simulink model "poly_Traj_lab"  (R2023b)
settings: Solver=VariableStepAuto  StartTime=0.0  StopTime=10.0  RelTol=1e-3
undefined symbols (not defined in the file or in its folder): X, Y, Z
libraries: sm_lib x16, nesl_utility x5, robotcorelib x2, robotmaniplib x1
settings Model: Creator=root  LastModifiedBy=root

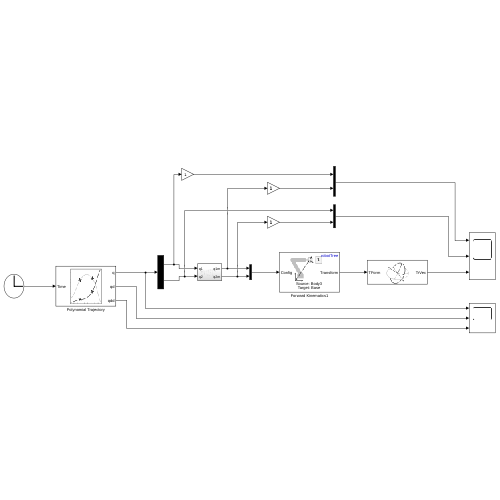
[thumbnail: Simulink's stored preview of the top-level diagram]
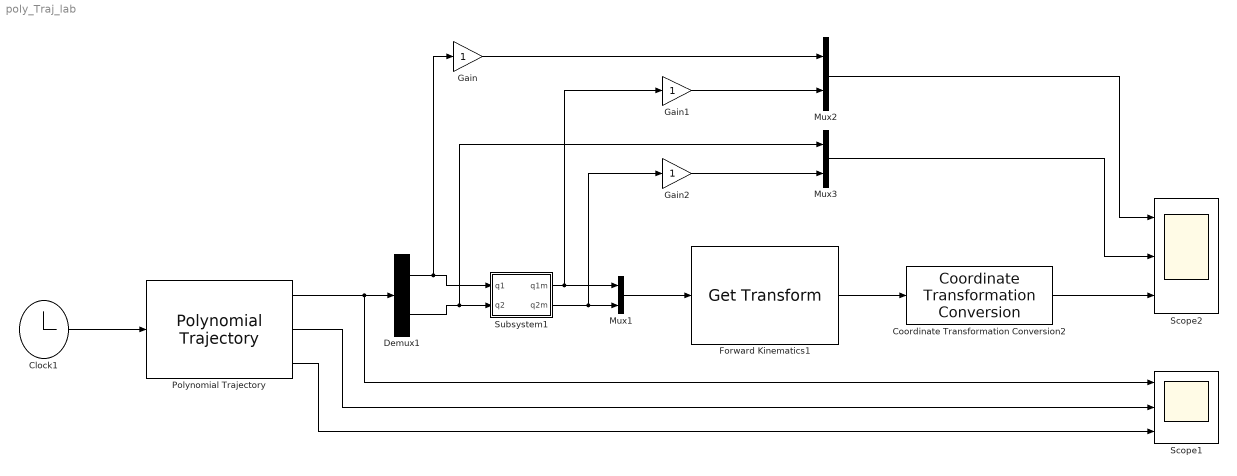
== system poly_Traj_lab ==
  Clock1 : Clock
  Coordinate Transformation Conversion2 : robotcorelib/Coordinate Transformation Conversion  InputRepresentation=Homogeneous Transformation  InputEulerSequence=ZYX  ShowTrVecInputPort=on  OutputRepresentation=Translation Vector  OutputEulerSequence=ZYX  ShowTrVecOutputPort=on  SimulateUsing=Interpreted execution
      settings: LibrarySourceBlock=navlib/Utilities/Coordinate Transformation Conversion
  Demux1 : Demux  Outputs=2
  Forward Kinematics1 : robotmaniplib/Get Transform  RigidBodyTree=robotTree  SourceBody=Body3  TargetBody=Base  SimulateUsing=Interpreted execution
  Gain : Gain
  Gain1 : Gain
  Gain2 : Gain
  Mux1 : Mux  Inputs=2
  Mux2 : Mux  Inputs=2
  Mux3 : Mux  Inputs=2
  Polynomial Trajectory : robotcorelib/Polynomial Trajectory  WaypointSource=Internal  Waypoints=[0 0 pi/2 pi/2; 0 0 -2*pi -2*pi]  TimePoints=[0 2 8 10]  TimeInterval=[ 1, 4 ]  Method=Cubic Polynomial  ParameterSource=Internal  VelocityBoundaryCondition=[0 0 0 0; 0 0 0 0]  AccelerationBoundaryCondition=zeros( 2, 5 )  SimulateUsing=Interpreted execution
  Scope1 : Scope  NumInputPorts=3
  Scope2 : Scope  NumInputPorts=3
  Subsystem1 : Subsystem
  wires:
  Polynomial Trajectory/2 -> Scope1/2
  Demux1/1 -> Gain/1, Subsystem1/1(q1)
  Forward Kinematics1/1 -> Coordinate Transformation Conversion2/1
  Demux1/2 -> Mux3/1, Subsystem1/2(q2)
  Clock1/1 -> Polynomial Trajectory/1
  Mux1/1 -> Forward Kinematics1/1
  Mux2/1 -> Scope2/1
  Coordinate Transformation Conversion2/1 -> Scope2/3
  Mux3/1 -> Scope2/2
  Gain2/1 -> Mux3/2
  Polynomial Trajectory/3 -> Scope1/3
  Subsystem1/2(q2m) -> Gain2/1, Mux1/2
  Gain/1 -> Mux2/1
  Gain1/1 -> Mux2/2
  Polynomial Trajectory/1 -> Scope1/1, Demux1/1
  Subsystem1/1(q1m) -> Gain1/1, Mux1/1

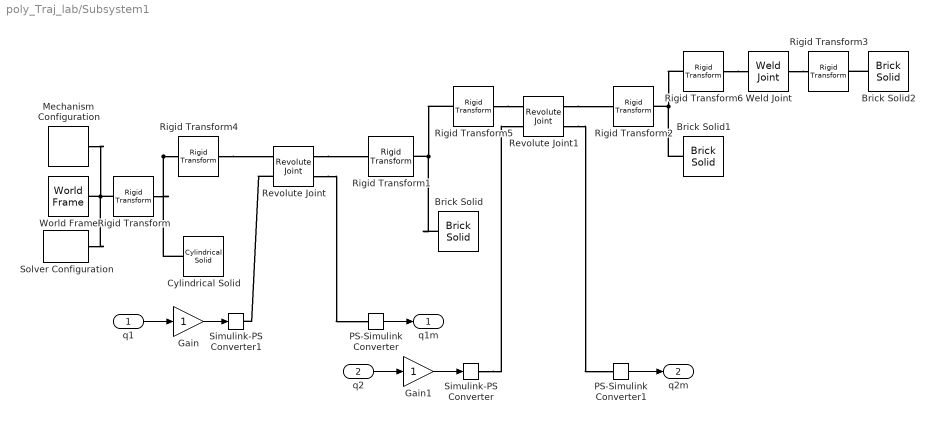
== system poly_Traj_lab/Subsystem1 ==
  q1 : Inport
  q2 : Inport  Port=2
  Brick Solid : sm_lib/Body Elements/Brick Solid  GraphicAmbientColor=[0.15 0.15 0.15 1.0]  BasedOnType=Density  BrickDimensions=[0.6 0.1 0.05]  BrickDimensionsUnits=m  CenterOfMass=[0 0 0]  CenterOfMassUnits=m  GraphicDiffuseColor=[1 0 0]  Density=1000  DensityUnits=kg/m^3  DoExposeReferenceFrame=on  GraphicEmissiveColor=[0.0 0.0 0.0 1.0]  ExportEntireGeometry=off  SerializedFrames=<Frames><Frame><Id>Frame1</Id><Value><Name>F1</Name><Origin><Source>GeometricFeature</Source><FeatureName>+x surface</FeatureName></Origin><PrimaryAxis><DefinedDirection>+Z</DefinedDirection><Source>ReferenceFrame</Source><SourceDirection>+Z</SourceDirection><FeatureName></FeatureName></PrimaryAxis><SecondaryAxis><DefinedDirection>+X</DefinedDirection><Source>ReferenceFrame</Source><SourceDirection>+X</SourceDirection><FeatureName></FeatureName></SecondaryAxis></Value></Frame></Frames>  MarkerShape=Sphere  MarkerSize=10  GraphicType=FromGeometry  InertiaType=CalculateFromGeometry  Mass=1  MassUnits=kg  MomentsOfInertia=[1 1 1]  MomentsOfInertiaUnits=kg*m^2  GraphicOpacity=1.0  ProductsOfInertia=[0 0 0]  ProductsOfInertiaUnits=kg*m^2  GraphicShininess=75  GraphicSpecularColor=[0.5 0.5 0.5 1.0]  GraphicVisPropType=SimpleVisualProperties
  Brick Solid1 : sm_lib/Body Elements/Brick Solid  GraphicAmbientColor=[0.15 0.15 0.15 1.0]  BasedOnType=Density  BrickDimensions=[0.4 0.1 0.05]  BrickDimensionsUnits=m  CenterOfMass=[0 0 0]  CenterOfMassUnits=m  GraphicDiffuseColor=[0 1 0]  Density=1000  DensityUnits=kg/m^3  DoExposeReferenceFrame=on  GraphicEmissiveColor=[0.0 0.0 0.0 1.0]  ExportEntireGeometry=off  SerializedFrames=<Frames><Frame><Id>Frame1</Id><Value><Name>F1</Name><Origin><Source>GeometricFeature</Source><FeatureName>+x surface</FeatureName></Origin><PrimaryAxis><DefinedDirection>+Z</DefinedDirection><Source>ReferenceFrame</Source><SourceDirection>+Z</SourceDirection><FeatureName></FeatureName></PrimaryAxis><SecondaryAxis><DefinedDirection>+X</DefinedDirection><Source>ReferenceFrame</Source><SourceDirection>+X</SourceDirection><FeatureName></FeatureName></SecondaryAxis></Value></Frame></Frames>  MarkerShape=Sphere  MarkerSize=10  GraphicType=FromGeometry  InertiaType=CalculateFromGeometry  Mass=1  MassUnits=kg  MomentsOfInertia=[1 1 1]  MomentsOfInertiaUnits=kg*m^2  GraphicOpacity=1.0  ProductsOfInertia=[0 0 0]  ProductsOfInertiaUnits=kg*m^2  GraphicShininess=75  GraphicSpecularColor=[0.5 0.5 0.5 1.0]  GraphicVisPropType=SimpleVisualProperties
  Brick Solid2 : sm_lib/Body Elements/Brick Solid  GraphicAmbientColor=[0.15 0.15 0.15 1.0]  BasedOnType=Density  BrickDimensions=[0.02 0.02 0.02]  BrickDimensionsUnits=m  CenterOfMass=[0 0 0]  CenterOfMassUnits=m  GraphicDiffuseColor=[1 0 1]  Density=1000  DensityUnits=kg/m^3  DoExposeReferenceFrame=on  GraphicEmissiveColor=[0.0 0.0 0.0 1.0]  ExportEntireGeometry=off  SerializedFrames=<Frames/>  MarkerShape=Sphere  MarkerSize=10  GraphicType=FromGeometry  InertiaType=CalculateFromGeometry  Mass=1  MassUnits=kg  MomentsOfInertia=[1 1 1]  MomentsOfInertiaUnits=kg*m^2  GraphicOpacity=1.0  ProductsOfInertia=[0 0 0]  ProductsOfInertiaUnits=kg*m^2  GraphicShininess=75  GraphicSpecularColor=[0.5 0.5 0.5 1.0]  GraphicVisPropType=SimpleVisualProperties
  Cylindrical Solid : sm_lib/Body Elements/Cylindrical Solid  GraphicAmbientColor=[0.15 0.15 0.15 1.0]  BasedOnType=Density  CenterOfMass=[0 0 0]  CenterOfMassUnits=m  GraphicDiffuseColor=[0 0 1]  CylinderLength=0.2  CylinderLengthUnits=m  CylinderRadius=0.05  CylinderRadiusUnits=m  Density=1000  DensityUnits=kg/m^3  DoExposeReferenceFrame=on  GraphicEmissiveColor=[0.0 0.0 0.0 1.0]  ExportEntireGeometry=off  SerializedFrames=<Frames><Frame><Id>Frame1</Id><Value><Name>F1</Name><Origin><Source>GeometricFeature</Source><FeatureName>top surface</FeatureName></Origin><PrimaryAxis><DefinedDirection>+Z</DefinedDirection><Source>ReferenceFrame</Source><SourceDirection>+Z</SourceDirection><FeatureName></FeatureName></PrimaryAxis><SecondaryAxis><DefinedDirection>+X</DefinedDirection><Source>ReferenceFrame</Source><SourceDirection>+X</SourceDirection><FeatureName></FeatureName></SecondaryAxis></Value></Frame></Frames>  MarkerShape=Sphere  MarkerSize=10  GraphicType=FromGeometry  InertiaType=CalculateFromGeometry  Mass=1  MassUnits=kg  MomentsOfInertia=[1 1 1]  MomentsOfInertiaUnits=kg*m^2  GraphicOpacity=1.0  ProductsOfInertia=[0 0 0]  ProductsOfInertiaUnits=kg*m^2  GraphicShininess=75  GraphicSpecularColor=[0.5 0.5 0.5 1.0]  GraphicVisPropType=SimpleVisualProperties
  Gain : Gain
  Gain1 : Gain
  Mechanism Configuration : sm_lib/Utilities/Mechanism Configuration  UniformGravity=Constant  GravityVector=[0 0 -9.80665]  GravityVectorUnits=m/s^2  LinearizationDelta=0.001  JointModeTransitionNonlinearIterations=2
  PS-Simulink Converter : nesl_utility/PS-Simulink Converter  PhysicalDomain=network_engine_domain  SubClassName=ps_output  LeftPortType=input  RightPortType=output  PseudoPeriodic=off  Frequencies=[]  VectorFormat=inherit  Unit=inherit  AffineConversion=off
  PS-Simulink Converter1 : nesl_utility/PS-Simulink Converter  PhysicalDomain=network_engine_domain  SubClassName=ps_output  LeftPortType=input  RightPortType=output  PseudoPeriodic=off  Frequencies=[]  VectorFormat=inherit  Unit=inherit  AffineConversion=off
  Revolute Joint : sm_lib/Joints/Revolute Joint  JointMode=Normal  SenseConstraintForce=off  SenseConstraintForceX=off  SenseConstraintForceY=off  SenseConstraintForceZ=off  SenseConstraintTorque=off  SenseConstraintTorqueX=off  SenseConstraintTorqueY=off  SenseConstraintTorqueZ=off  SenseTotalForce=off  SenseTotalForceX=off  SenseTotalForceY=off  SenseTotalForceZ=off  SenseTotalTorque=off  SenseTotalTorqueX=off  SenseTotalTorqueY=off  SenseTotalTorqueZ=off  CompositeWrenchDir=FollowerOnBase  CompositeWrenchFrame=BaseFrame  EquilibriumPosition=0  EquilibriumPositionUnits=deg  SpringStiffness=0  SpringStiffnessUnits=N*m/deg  DampingCoefficient=0  DampingCoefficientUnits=N*m/(deg/s)  TorqueActuationMode=ComputedTorque  MotionActuationMode=InputMotion  SensePosition=on  SenseVelocity=off  SenseAcceleration=off  SenseTorqueForce=off  SenseLowerLimitTorqueForce=off  SenseUpperLimitTorqueForce=off  LowerLimitSpecify=off  LowerLimitBound=-90  LowerLimitBoundUnits=deg  LowerLimitStiffness=1e4  LowerLimitStiffnessUnits=N*m/deg  LowerLimitDamping=10  LowerLimitDampingUnits=N*m/(deg/s)  LowerLimitTransitionRegionWidth=0.1  LowerLimitTransitionRegionWidthUnits=deg  UpperLimitSpecify=off  UpperLimitBound=90  UpperLimitBoundUnits=deg  UpperLimitStiffness=1e4  UpperLimitStiffnessUnits=N*m/deg  UpperLimitDamping=10  UpperLimitDampingUnits=N*m/(deg/s)  UpperLimitTransitionRegionWidth=0.1  UpperLimitTransitionRegionWidthUnits=deg  PositionTargetSpecify=off  PositionTargetPriority=High  PositionTargetValue=0  PositionTargetValueUnits=deg  VelocityTargetSpecify=off  VelocityTargetPriority=High  VelocityTargetValue=0  VelocityTargetValueUnits=deg/s
  Revolute Joint1 : sm_lib/Joints/Revolute Joint  JointMode=Normal  SenseConstraintForce=off  SenseConstraintForceX=off  SenseConstraintForceY=off  SenseConstraintForceZ=off  SenseConstraintTorque=off  SenseConstraintTorqueX=off  SenseConstraintTorqueY=off  SenseConstraintTorqueZ=off  SenseTotalForce=off  SenseTotalForceX=off  SenseTotalForceY=off  SenseTotalForceZ=off  SenseTotalTorque=off  SenseTotalTorqueX=off  SenseTotalTorqueY=off  SenseTotalTorqueZ=off  CompositeWrenchDir=FollowerOnBase  CompositeWrenchFrame=BaseFrame  EquilibriumPosition=0  EquilibriumPositionUnits=deg  SpringStiffness=0  SpringStiffnessUnits=N*m/deg  DampingCoefficient=0  DampingCoefficientUnits=N*m/(deg/s)  TorqueActuationMode=ComputedTorque  MotionActuationMode=InputMotion  SensePosition=on  SenseVelocity=off  SenseAcceleration=off  SenseTorqueForce=off  SenseLowerLimitTorqueForce=off  SenseUpperLimitTorqueForce=off  LowerLimitSpecify=off  LowerLimitBound=-90  LowerLimitBoundUnits=deg  LowerLimitStiffness=1e4  LowerLimitStiffnessUnits=N*m/deg  LowerLimitDamping=10  LowerLimitDampingUnits=N*m/(deg/s)  LowerLimitTransitionRegionWidth=0.1  LowerLimitTransitionRegionWidthUnits=deg  UpperLimitSpecify=off  UpperLimitBound=90  UpperLimitBoundUnits=deg  UpperLimitStiffness=1e4  UpperLimitStiffnessUnits=N*m/deg  UpperLimitDamping=10  UpperLimitDampingUnits=N*m/(deg/s)  UpperLimitTransitionRegionWidth=0.1  UpperLimitTransitionRegionWidthUnits=deg  PositionTargetSpecify=off  PositionTargetPriority=High  PositionTargetValue=0  PositionTargetValueUnits=deg  VelocityTargetSpecify=off  VelocityTargetPriority=High  VelocityTargetValue=0  VelocityTargetValueUnits=deg/s
  Rigid Transform : sm_lib/Frames and Transforms/Rigid Transform  TranslationMethod=Cartesian  TranslationStandardOffset=0  TranslationStandardOffsetUnits=m  TranslationStandardAxis=+Z  TranslationCartesianOffset=[0 0 0.1]  TranslationCartesianOffsetUnits=m  TranslationROffset=0  TranslationROffsetUnits=m  TranslationZOffset=0  TranslationZOffsetUnits=m  TranslationThetaOffset=0  TranslationThetaOffsetUnits=deg  RotationMethod=None  RotationAngleUnits=deg  RotationStandardAxis=+Z  RotationAngle=0.0  RotationArbitraryAxis=[0 0 1]  FollAlignAxisA=+X  BaseAlignAxisA=+Y  FollAlignAxisB=+Y  BaseAlignAxisB=+Z  RotationSequenceAxes=FollowerAxes  RotationSequence=XYX  RotationSequenceAngles=[0 0 0]  RotationSequenceAnglesUnits=deg  RotationMatrix=[1 0 0; 0 1 0; 0 0 1]  Quaternion=[1 0 0 0]
  Rigid Transform1 : sm_lib/Frames and Transforms/Rigid Transform  TranslationMethod=Cartesian  TranslationStandardOffset=0  TranslationStandardOffsetUnits=m  TranslationStandardAxis=+Z  TranslationCartesianOffset=[0.3 0 0.025]  TranslationCartesianOffsetUnits=m  TranslationROffset=0  TranslationROffsetUnits=m  TranslationZOffset=0  TranslationZOffsetUnits=m  TranslationThetaOffset=0  TranslationThetaOffsetUnits=deg  RotationMethod=None  RotationAngleUnits=deg  RotationStandardAxis=+Z  RotationAngle=0.0  RotationArbitraryAxis=[0 0 1]  FollAlignAxisA=+X  BaseAlignAxisA=+Y  FollAlignAxisB=+Y  BaseAlignAxisB=+Z  RotationSequenceAxes=FollowerAxes  RotationSequence=XYX  RotationSequenceAngles=[0 0 0]  RotationSequenceAnglesUnits=deg  RotationMatrix=[1 0 0; 0 1 0; 0 0 1]  Quaternion=[1 0 0 0]
  Rigid Transform2 : sm_lib/Frames and Transforms/Rigid Transform  TranslationMethod=Cartesian  TranslationStandardOffset=0  TranslationStandardOffsetUnits=m  TranslationStandardAxis=+Z  TranslationCartesianOffset=[0.2 0 0.025]  TranslationCartesianOffsetUnits=m  TranslationROffset=0  TranslationROffsetUnits=m  TranslationZOffset=0  TranslationZOffsetUnits=m  TranslationThetaOffset=0  TranslationThetaOffsetUnits=deg  RotationMethod=None  RotationAngleUnits=deg  RotationStandardAxis=+Z  RotationAngle=0.0  RotationArbitraryAxis=[0 0 1]  FollAlignAxisA=+X  BaseAlignAxisA=+Y  FollAlignAxisB=+Y  BaseAlignAxisB=+Z  RotationSequenceAxes=FollowerAxes  RotationSequence=XYX  RotationSequenceAngles=[0 0 0]  RotationSequenceAnglesUnits=deg  RotationMatrix=[1 0 0; 0 1 0; 0 0 1]  Quaternion=[1 0 0 0]
  Rigid Transform3 : sm_lib/Frames and Transforms/Rigid Transform  TranslationMethod=Cartesian  TranslationStandardOffset=0  TranslationStandardOffsetUnits=m  TranslationStandardAxis=+Z  TranslationCartesianOffset=[0.01 0 0]  TranslationCartesianOffsetUnits=m  TranslationROffset=0  TranslationROffsetUnits=m  TranslationZOffset=0  TranslationZOffsetUnits=m  TranslationThetaOffset=0  TranslationThetaOffsetUnits=deg  RotationMethod=None  RotationAngleUnits=deg  RotationStandardAxis=+Z  RotationAngle=0.0  RotationArbitraryAxis=[0 0 1]  FollAlignAxisA=+X  BaseAlignAxisA=+Y  FollAlignAxisB=+Y  BaseAlignAxisB=+Z  RotationSequenceAxes=FollowerAxes  RotationSequence=XYX  RotationSequenceAngles=[0 0 0]  RotationSequenceAnglesUnits=deg  RotationMatrix=[1 0 0; 0 1 0; 0 0 1]  Quaternion=[1 0 0 0]
  Rigid Transform4 : sm_lib/Frames and Transforms/Rigid Transform  TranslationMethod=Cartesian  TranslationStandardOffset=0  TranslationStandardOffsetUnits=m  TranslationStandardAxis=+Z  TranslationCartesianOffset=[0 0 0.1]  TranslationCartesianOffsetUnits=m  TranslationROffset=0  TranslationROffsetUnits=m  TranslationZOffset=0  TranslationZOffsetUnits=m  TranslationThetaOffset=0  TranslationThetaOffsetUnits=deg  RotationMethod=None  RotationAngleUnits=deg  RotationStandardAxis=+Z  RotationAngle=0.0  RotationArbitraryAxis=[0 0 1]  FollAlignAxisA=+X  BaseAlignAxisA=+Y  FollAlignAxisB=+Y  BaseAlignAxisB=+Z  RotationSequenceAxes=FollowerAxes  RotationSequence=XYX  RotationSequenceAngles=[0 0 0]  RotationSequenceAnglesUnits=deg  RotationMatrix=[1 0 0; 0 1 0; 0 0 1]  Quaternion=[1 0 0 0]
  Rigid Transform5 : sm_lib/Frames and Transforms/Rigid Transform  TranslationMethod=Cartesian  TranslationStandardOffset=0  TranslationStandardOffsetUnits=m  TranslationStandardAxis=+Z  TranslationCartesianOffset=[0.3 0 0.025]  TranslationCartesianOffsetUnits=m  TranslationROffset=0  TranslationROffsetUnits=m  TranslationZOffset=0  TranslationZOffsetUnits=m  TranslationThetaOffset=0  TranslationThetaOffsetUnits=deg  RotationMethod=None  RotationAngleUnits=deg  RotationStandardAxis=+Z  RotationAngle=0.0  RotationArbitraryAxis=[0 0 1]  FollAlignAxisA=+X  BaseAlignAxisA=+Y  FollAlignAxisB=+Y  BaseAlignAxisB=+Z  RotationSequenceAxes=FollowerAxes  RotationSequence=XYX  RotationSequenceAngles=[0 0 0]  RotationSequenceAnglesUnits=deg  RotationMatrix=[1 0 0; 0 1 0; 0 0 1]  Quaternion=[1 0 0 0]
  Rigid Transform6 : sm_lib/Frames and Transforms/Rigid Transform  TranslationMethod=Cartesian  TranslationStandardOffset=0  TranslationStandardOffsetUnits=m  TranslationStandardAxis=+Z  TranslationCartesianOffset=[0.2 0 0]  TranslationCartesianOffsetUnits=m  TranslationROffset=0  TranslationROffsetUnits=m  TranslationZOffset=0  TranslationZOffsetUnits=m  TranslationThetaOffset=0  TranslationThetaOffsetUnits=deg  RotationMethod=None  RotationAngleUnits=deg  RotationStandardAxis=+Z  RotationAngle=0.0  RotationArbitraryAxis=[0 0 1]  FollAlignAxisA=+X  BaseAlignAxisA=+Y  FollAlignAxisB=+Y  BaseAlignAxisB=+Z  RotationSequenceAxes=FollowerAxes  RotationSequence=XYX  RotationSequenceAngles=[0 0 0]  RotationSequenceAnglesUnits=deg  RotationMatrix=[1 0 0; 0 1 0; 0 0 1]  Quaternion=[1 0 0 0]
  Simulink-PS Converter : nesl_utility/Simulink-PS Converter  PhysicalDomain=network_engine_domain  SubClassName=ps_input  LeftPortType=input  RightPortType=output  PseudoPeriodic=off  Frequencies=[]  NoiseDistribution=none  NoiseParameters=[]  Unit=1  AffineConversion=off  FilteringAndDerivatives=filter  SimscapeFilterOrder=2  InputFilterTimeConstant=0.001  UdotUserProvided=0
  Simulink-PS Converter1 : nesl_utility/Simulink-PS Converter  PhysicalDomain=network_engine_domain  SubClassName=ps_input  LeftPortType=input  RightPortType=output  PseudoPeriodic=off  Frequencies=[]  NoiseDistribution=none  NoiseParameters=[]  Unit=1  AffineConversion=off  FilteringAndDerivatives=filter  SimscapeFilterOrder=2  InputFilterTimeConstant=0.001  UdotUserProvided=0
  Solver Configuration : nesl_utility/Solver Configuration  PhysicalDomain=network_engine_domain  SubClassName=solver  LeftPortType=input  RightPortType=generic  Tones=[]  Harmonics=[]  SimulateNoise=off  Profile=off  UseLocalSampling=off  EnableSwitchedLinearOptims=on  FrequencyDomain=off  UseCCode=off  RelTol=0.001  AbsTol=0.001  MinStep=1e-09  ToWorkspace=off  RevertToSquareIcSolve=off  NumHomotopyIterations=100  PhasorMode=off  PhasorModeNumHarmonics=1  ConsistencySolver=NEWTON_XTOL_AFTER_FTOL  IndexReductionMethod=DerivativeReplacement  DoDC=off  ResidualTolerance=1e-09  ConsistencyTolSource=GLOBAL  ConsistencyAbsTol=0.001  ConsistencyRelTol=0.001  ConsistencyTolFactor=0.001  UseLocalSolver=off  LocalSolverChoice=NE_BACKWARD_EULER_ADVANCER  ResolveIndetEquations=on  FunctionEvalNumThread=1  LocalSolverSampleTime=0.001  DoFixedCost=off  MaxNonlinIter=3  MaxModeIter=2  ComputeImpulses=off  ImpulseIterations=2  LinearAlgebra=auto  LinearAlgebraNumThread=0  EquationFormulation=NE_TIME_EF  DelaysMemoryBudget=1024  AutomaticFiltering=on  FilteringTimeConstant=0.001  PartitionStorageMethod=AS_NEEDED  PartitionMemoryBudget=1024  PartitionMethod=ROBUST  MultibodyUseLocalSolver=off  MultibodyLocalSolverChoice=ODE1  MultibodyLocalSolverSampleTime=0.001
  Weld Joint : sm_lib/Joints/Weld Joint  JointMode=Normal  SenseConstraintForce=off  SenseConstraintForceX=off  SenseConstraintForceY=off  SenseConstraintForceZ=off  SenseConstraintTorque=off  SenseConstraintTorqueX=off  SenseConstraintTorqueY=off  SenseConstraintTorqueZ=off  SenseTotalForce=off  SenseTotalForceX=off  SenseTotalForceY=off  SenseTotalForceZ=off  SenseTotalTorque=off  SenseTotalTorqueX=off  SenseTotalTorqueY=off  SenseTotalTorqueZ=off  CompositeWrenchDir=FollowerOnBase  CompositeWrenchFrame=BaseFrame
  World Frame : sm_lib/Frames and Transforms/World Frame
  q1m : Outport
  q2m : Outport  Port=2
  wires:
  Gain1/1 -> Simulink-PS Converter/1
  Gain/1 -> Simulink-PS Converter1/1
  PS-Simulink Converter/1 -> q1m/1
  PS-Simulink Converter1/1 -> q2m/1
  q2/1 -> Gain1/1
  q1/1 -> Gain/1
  connections:
  Brick Solid/RConn1 -- Rigid Transform5/LConn1 -- Rigid Transform1/RConn1
  Rigid Transform4/LConn1 -- Cylindrical Solid/RConn1 -- Rigid Transform/RConn1
  Rigid Transform6/LConn1 -- Brick Solid1/RConn1 -- Rigid Transform2/RConn1
  Solver Configuration/RConn1 -- Mechanism Configuration/RConn1 -- Rigid Transform/LConn1 -- World Frame/RConn1
  Revolute Joint/LConn2 -- Simulink-PS Converter1/RConn1
  Rigid Transform4/RConn1 -- Revolute Joint/LConn1
  Rigid Transform5/RConn1 -- Revolute Joint1/LConn1
  Revolute Joint/RConn1 -- Rigid Transform1/LConn1
  Revolute Joint/RConn2 -- PS-Simulink Converter/LConn1
  Weld Joint/RConn1 -- Rigid Transform3/LConn1
  Brick Solid2/RConn1 -- Rigid Transform3/RConn1
  Simulink-PS Converter/RConn1 -- Revolute Joint1/LConn2
  Revolute Joint1/RConn2 -- PS-Simulink Converter1/LConn1
  Rigid Transform6/RConn1 -- Weld Joint/LConn1
  Revolute Joint1/RConn1 -- Rigid Transform2/LConn1
